simulink model "greenbotics_state_machine"  (R2026b)
settings: Solver=FixedStepDiscrete  StopTime=13.96666667  FixedStep=1/30
settings Model: Creator=rakshith  LastModifiedBy=rakshith
settings DataIOCC: SaveFormat=Array

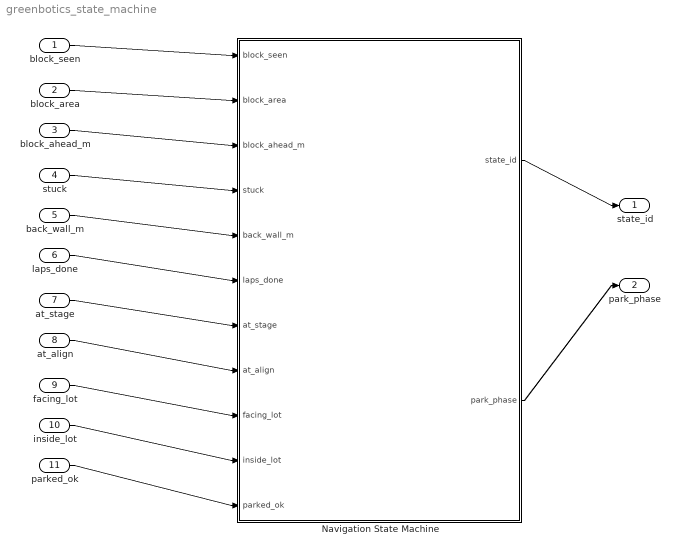
== system greenbotics_state_machine ==
  block_seen : Inport  OutDataTypeStr=double  PortDimensions=1  SampleTime=1/30
  block_area : Inport  Port=2  OutDataTypeStr=double  PortDimensions=1  SampleTime=1/30
  block_ahead_m : Inport  Port=3  OutDataTypeStr=double  PortDimensions=1  SampleTime=1/30
  stuck : Inport  Port=4  OutDataTypeStr=double  PortDimensions=1  SampleTime=1/30
  back_wall_m : Inport  Port=5  OutDataTypeStr=double  PortDimensions=1  SampleTime=1/30
  laps_done : Inport  Port=6  OutDataTypeStr=double  PortDimensions=1  SampleTime=1/30
  at_stage : Inport  Port=7  OutDataTypeStr=double  PortDimensions=1  SampleTime=1/30
  at_align : Inport  Port=8  OutDataTypeStr=double  PortDimensions=1  SampleTime=1/30
  facing_lot : Inport  Port=9  OutDataTypeStr=double  PortDimensions=1  SampleTime=1/30
  inside_lot : Inport  Port=10  OutDataTypeStr=double  PortDimensions=1  SampleTime=1/30
  parked_ok : Inport  Port=11  OutDataTypeStr=double  PortDimensions=1  SampleTime=1/30
  Navigation State Machine : Stateflow chart  TreatAsAtomicUnit=on
  state_id : Outport
  park_phase : Outport  Port=2
  wires:
  block_seen/1 -> Navigation State Machine/1(block_seen)
  block_area/1 -> Navigation State Machine/2(block_area)
  block_ahead_m/1 -> Navigation State Machine/3(block_ahead_m)
  stuck/1 -> Navigation State Machine/4(stuck)
  back_wall_m/1 -> Navigation State Machine/5(back_wall_m)
  laps_done/1 -> Navigation State Machine/6(laps_done)
  at_stage/1 -> Navigation State Machine/7(at_stage)
  at_align/1 -> Navigation State Machine/8(at_align)
  facing_lot/1 -> Navigation State Machine/9(facing_lot)
  inside_lot/1 -> Navigation State Machine/10(inside_lot)
  parked_ok/1 -> Navigation State Machine/11(parked_ok)
  Navigation State Machine/1(state_id) -> state_id/1
  Navigation State Machine/2(park_phase) -> park_phase/1

== stateflow chart greenbotics_state_machine/Navigation State Machine ==
  state DRIVE
    entry: park_phase = 0;
    during: cooldown = max(0, cooldown - 1);
    state DRIVING_STRAIGHT
      entry: state_id = 1;
    state AVOIDING_BLOCK
      entry: state_id = 2;
    state CLEARING
      entry: state_id = 3; frames_lost = 0;
      during: frames_lost = frames_lost + 1;
    (default) -> DRIVING_STRAIGHT
    DRIVING_STRAIGHT -> AVOIDING_BLOCK : [block_seen > 0.5 && block_area > MIN_AREA]
    CLEARING -> DRIVING_STRAIGHT [order 2] : [frames_lost >= CLEARANCE_FRAMES]
    CLEARING -> AVOIDING_BLOCK [order 1] : [block_seen > 0.5]
    AVOIDING_BLOCK -> CLEARING : [block_seen < 0.5]
  state EMERGENCY_REVERSE
    entry: state_id = 4; emerg_frames = 0;
    during: emerg_frames = emerg_frames + 1;
    exit: cooldown = COOLDOWN_FRAMES;
  state PARK
    entry: state_id = 5;
    state APPROACH
      entry: park_phase = 1;
    state ALIGN
      entry: park_phase = 2;
    state TURN_IN
      entry: park_phase = 3;
    state ENTER
      entry: park_phase = 4;
    state STRAIGHTEN
      entry: park_phase = 5; park_timer = 0;
      during: park_timer = park_timer + 1;
    (default) -> APPROACH
    APPROACH -> ALIGN : [at_stage > 0.5]
    ALIGN -> TURN_IN : [at_align > 0.5]
    TURN_IN -> ENTER : [facing_lot > 0.5]
    ENTER -> STRAIGHTEN : [inside_lot > 0.5]
  state MISSION_COMPLETE
    entry: state_id = 6;
  (default) -> DRIVE
  DRIVE -> EMERGENCY_REVERSE [order 2] : [stuck > 0.5 || (block_ahead_m < EMERG_DIST_M && cooldown <= 0)]
  EMERGENCY_REVERSE -> DRIVE : [emerg_frames >= REVERSE_FRAMES || back_wall_m < BACK_WALL_MIN_M]
  DRIVE -> PARK [order 1] : [laps_done >= 3]
  STRAIGHTEN -> MISSION_COMPLETE : [parked_ok > 0.5 || park_timer > PARK_TIMEOUT]
  data: block_seen input double size=1; block_area input double size=1; block_ahead_m input double size=1; stuck input double size=1; back_wall_m input double size=1; laps_done input double size=1; at_stage input double size=1; at_align input double size=1; facing_lot input double size=1; inside_lot input double size=1; parked_ok input double size=1; state_id output double size=1 =0; park_phase output double size=1 =0; frames_lost local double size=1 =0; emerg_frames local double size=1 =0; cooldown local double size=1 =0; park_timer local double size=1 =0; MIN_AREA constant double size=1 =1500; CLEARANCE_FRAMES constant double size=1 =45; EMERG_DIST_M constant double size=1 =0.19; BACK_WALL_MIN_M constant double size=1 =0.22; REVERSE_FRAMES constant double size=1 =24; COOLDOWN_FRAMES constant double size=1 =45; PARK_TIMEOUT constant double size=1 =150
